simulink model "ASM_Traffic_new"  (R2024a)
settings: Solver=ode1  StartTime=SIM.tstart.v  StopTime=SIM.tend.v  FixedStep=SIM.StepSize.v  RelTol=1e-3
PostLoadFcn:
  | if any(exist('dsrtsu_mdlpostloadfcn', 'file') ~= 0), dsrtsu_mdlpostloadfcn('Execute', bdroot); end
  | try, asm_mdl_postloadfcn(bdroot, 'UpdateModel', 3600); catch, disp(lasterr); end,
InitFcn:
  | , if any(exist('rtifpga_mdlclblib', 'file') ~= 0), rtifpga_mdlclblib('Init', bdroot); end,
  | , if any(exist('dsmpb_private', 'file') ~= 0), dsmpb_private('dsmpb_mdlclblib', 'Init', bdroot); end,
undefined symbols (not defined in the file): _to_, a0b2, ASM_BrakeHydraulics_DemoSystems, ASM_VehicleDynamics_DemoSystems, b98103fe8ad365046cd0, BrakeCircuit, CPT, Crankshaft, DiscIntNeverNeededParam, dsmsi, FinalDriveAssembly, MDL, ModeSignals, Pos_BrakePedal_Maneuver, rad, RefSignals, s_to_rpm, SIM, SoftECU, Suspension, Tire, Transmission
libraries: ASM_Traffic_lib x135, simulink x100, ASM_Utils_lib x77, ASM_VehicleDynamics_lib x70, ASM_Environment_lib x22, dsmpblib x20, dsmsilib x15, MDLD_Utils_lib x10, ASM_BrakeHydraulics_lib x3
(part 17 of 63)

== system ASM_Traffic_new/AnimationInterface/ANIMATION_INTERFACE/Bounding_Boxes/BoundingBox_4 ==
  Index[] : Inport
  BoundigBoxes_Animation : Inport  Port=2
  Bus Selector : BusSelector  OutputSignals=Pos_x_CoorSysE[m],Pos_y_CoorSysE[m],Pos_z_CoorSysE[m],Angle_z_Objects_CoorSysE[deg],Angle_y_Objects_CoorSysE[deg],Angle_x_Objects_CoorSysE[deg],Length_Object[m],Width_Object[m],Height_Object[m]
  Mux : Mux  Inputs=3
  Mux1 : Mux  Inputs=3
  Mux2 : Mux  Inputs=3
  Selector{1..9} (9 alike) : Selector  IndexOptions=Index vector (port)  Indices=[1 3]  OutputSizes=1
  Pos_CoorSysE[m] : Outport  VectorParamsAs1DForOutWhenUnconnected=off
  Angle_CoorSysE[m] : Outport  Port=2  VectorParamsAs1DForOutWhenUnconnected=off
  Dimensions[m] : Outport  Port=3  VectorParamsAs1DForOutWhenUnconnected=off
  wires:
  Bus Selector/9 -> Selector9/1  "<Height_Object[m]>"
  Bus Selector/8 -> Selector8/1  "<Width_Object[m]>"
  Bus Selector/7 -> Selector6/1  "<Length_Object[m]>"
  Bus Selector/6 -> Selector7/1  "<Angle_x_Objects_CoorSysE[deg]>"
  Bus Selector/5 -> Selector5/1  "<Angle_y_Objects_CoorSysE[deg]>"
  Bus Selector/4 -> Selector4/1  "<Angle_z_Objects_CoorSysE[deg]>"
  Bus Selector/3 -> Selector3/1  "<Pos_z_CoorSysE[m]>"
  Bus Selector/2 -> Selector2/1  "<Pos_y_CoorSysE[m]>"
  Bus Selector/1 -> Selector1/1  "<Pos_x_CoorSysE[m]>"
  BoundigBoxes_Animation/1 -> Bus Selector/1
  Selector5/1 -> Mux1/2
  Mux1/1 -> Angle_CoorSysE[m]/1
  Mux/1 -> Pos_CoorSysE[m]/1
  Index[]/1 -> Selector3/2, Selector4/2, Selector9/2, Selector8/2, Selector6/2, Selector7/2, Selector5/2, Selector2/2, Selector1/2
  Selector1/1 -> Mux/1
  Selector2/1 -> Mux/2
  Selector3/1 -> Mux/3
  Selector7/1 -> Mux1/3
  Selector4/1 -> Mux1/1
  Selector6/1 -> Mux2/1
  Selector8/1 -> Mux2/2
  Selector9/1 -> Mux2/3
  Mux2/1 -> Dimensions[m]/1

== system ASM_Traffic_new/AnimationInterface/ANIMATION_INTERFACE/Bounding_Boxes/BoundingBox_5 ==
  Index[] : Inport
  BoundigBoxes_Animation : Inport  Port=2
  Bus Selector : BusSelector  OutputSignals=Pos_x_CoorSysE[m],Pos_y_CoorSysE[m],Pos_z_CoorSysE[m],Angle_z_Objects_CoorSysE[deg],Angle_y_Objects_CoorSysE[deg],Angle_x_Objects_CoorSysE[deg],Length_Object[m],Width_Object[m],Height_Object[m]
  Mux : Mux  Inputs=3
  Mux1 : Mux  Inputs=3
  Mux2 : Mux  Inputs=3
  Selector{1..9} (9 alike) : Selector  IndexOptions=Index vector (port)  Indices=[1 3]  OutputSizes=1
  Pos_CoorSysE[m] : Outport  VectorParamsAs1DForOutWhenUnconnected=off
  Angle_CoorSysE[m] : Outport  Port=2  VectorParamsAs1DForOutWhenUnconnected=off
  Dimensions[m] : Outport  Port=3  VectorParamsAs1DForOutWhenUnconnected=off
  wires:
  Mux2/1 -> Dimensions[m]/1
  Selector9/1 -> Mux2/3
  Selector8/1 -> Mux2/2
  Selector6/1 -> Mux2/1
  Selector4/1 -> Mux1/1
  Selector7/1 -> Mux1/3
  Selector3/1 -> Mux/3
  Selector2/1 -> Mux/2
  Selector1/1 -> Mux/1
  Index[]/1 -> Selector1/2, Selector2/2, Selector5/2, Selector7/2, Selector6/2, Selector8/2, Selector9/2, Selector4/2, Selector3/2
  Mux/1 -> Pos_CoorSysE[m]/1
  Mux1/1 -> Angle_CoorSysE[m]/1
  Selector5/1 -> Mux1/2
  BoundigBoxes_Animation/1 -> Bus Selector/1
  Bus Selector/1 -> Selector1/1  "<Pos_x_CoorSysE[m]>"
  Bus Selector/2 -> Selector2/1  "<Pos_y_CoorSysE[m]>"
  Bus Selector/3 -> Selector3/1  "<Pos_z_CoorSysE[m]>"
  Bus Selector/4 -> Selector4/1  "<Angle_z_Objects_CoorSysE[deg]>"
  Bus Selector/5 -> Selector5/1  "<Angle_y_Objects_CoorSysE[deg]>"
  Bus Selector/6 -> Selector7/1  "<Angle_x_Objects_CoorSysE[deg]>"
  Bus Selector/7 -> Selector6/1  "<Length_Object[m]>"
  Bus Selector/8 -> Selector8/1  "<Width_Object[m]>"
  Bus Selector/9 -> Selector9/1  "<Height_Object[m]>"

== system ASM_Traffic_new/AnimationInterface/ANIMATION_INTERFACE/Bounding_Boxes/BoundingBox_6 ==
  Index[] : Inport
  BoundigBoxes_Animation : Inport  Port=2
  Bus Selector : BusSelector  OutputSignals=Pos_x_CoorSysE[m],Pos_y_CoorSysE[m],Pos_z_CoorSysE[m],Angle_z_Objects_CoorSysE[deg],Angle_y_Objects_CoorSysE[deg],Angle_x_Objects_CoorSysE[deg],Length_Object[m],Width_Object[m],Height_Object[m]
  Mux : Mux  Inputs=3
  Mux1 : Mux  Inputs=3
  Mux2 : Mux  Inputs=3
  Selector{1..9} (9 alike) : Selector  IndexOptions=Index vector (port)  Indices=[1 3]  OutputSizes=1
  Pos_CoorSysE[m] : Outport  VectorParamsAs1DForOutWhenUnconnected=off
  Angle_CoorSysE[m] : Outport  Port=2  VectorParamsAs1DForOutWhenUnconnected=off
  Dimensions[m] : Outport  Port=3  VectorParamsAs1DForOutWhenUnconnected=off
  wires:
  Bus Selector/9 -> Selector9/1  "<Height_Object[m]>"
  Bus Selector/8 -> Selector8/1  "<Width_Object[m]>"
  Bus Selector/7 -> Selector6/1  "<Length_Object[m]>"
  Bus Selector/6 -> Selector7/1  "<Angle_x_Objects_CoorSysE[deg]>"
  Bus Selector/5 -> Selector5/1  "<Angle_y_Objects_CoorSysE[deg]>"
  Bus Selector/4 -> Selector4/1  "<Angle_z_Objects_CoorSysE[deg]>"
  Bus Selector/3 -> Selector3/1  "<Pos_z_CoorSysE[m]>"
  Bus Selector/2 -> Selector2/1  "<Pos_y_CoorSysE[m]>"
  Bus Selector/1 -> Selector1/1  "<Pos_x_CoorSysE[m]>"
  BoundigBoxes_Animation/1 -> Bus Selector/1
  Selector5/1 -> Mux1/2
  Mux1/1 -> Angle_CoorSysE[m]/1
  Mux/1 -> Pos_CoorSysE[m]/1
  Index[]/1 -> Selector3/2, Selector4/2, Selector9/2, Selector8/2, Selector6/2, Selector7/2, Selector5/2, Selector2/2, Selector1/2
  Selector1/1 -> Mux/1
  Selector2/1 -> Mux/2
  Selector3/1 -> Mux/3
  Selector7/1 -> Mux1/3
  Selector4/1 -> Mux1/1
  Selector6/1 -> Mux2/1
  Selector8/1 -> Mux2/2
  Selector9/1 -> Mux2/3
  Mux2/1 -> Dimensions[m]/1

== system ASM_Traffic_new/AnimationInterface/ANIMATION_INTERFACE/Bounding_Boxes/BoundingBox_7 ==
  Index[] : Inport
  BoundigBoxes_Animation : Inport  Port=2
  Bus Selector : BusSelector  OutputSignals=Pos_x_CoorSysE[m],Pos_y_CoorSysE[m],Pos_z_CoorSysE[m],Angle_z_Objects_CoorSysE[deg],Angle_y_Objects_CoorSysE[deg],Angle_x_Objects_CoorSysE[deg],Length_Object[m],Width_Object[m],Height_Object[m]
  Mux : Mux  Inputs=3
  Mux1 : Mux  Inputs=3
  Mux2 : Mux  Inputs=3
  Selector{1..9} (9 alike) : Selector  IndexOptions=Index vector (port)  Indices=[1 3]  OutputSizes=1
  Pos_CoorSysE[m] : Outport  VectorParamsAs1DForOutWhenUnconnected=off
  Angle_CoorSysE[m] : Outport  Port=2  VectorParamsAs1DForOutWhenUnconnected=off
  Dimensions[m] : Outport  Port=3  VectorParamsAs1DForOutWhenUnconnected=off
  wires:
  Bus Selector/9 -> Selector9/1  "<Height_Object[m]>"
  Bus Selector/8 -> Selector8/1  "<Width_Object[m]>"
  Bus Selector/7 -> Selector6/1  "<Length_Object[m]>"
  Bus Selector/6 -> Selector7/1  "<Angle_x_Objects_CoorSysE[deg]>"
  Bus Selector/5 -> Selector5/1  "<Angle_y_Objects_CoorSysE[deg]>"
  Bus Selector/4 -> Selector4/1  "<Angle_z_Objects_CoorSysE[deg]>"
  Bus Selector/3 -> Selector3/1  "<Pos_z_CoorSysE[m]>"
  Bus Selector/2 -> Selector2/1  "<Pos_y_CoorSysE[m]>"
  Bus Selector/1 -> Selector1/1  "<Pos_x_CoorSysE[m]>"
  BoundigBoxes_Animation/1 -> Bus Selector/1
  Selector5/1 -> Mux1/2
  Mux1/1 -> Angle_CoorSysE[m]/1
  Mux/1 -> Pos_CoorSysE[m]/1
  Index[]/1 -> Selector3/2, Selector4/2, Selector9/2, Selector8/2, Selector6/2, Selector7/2, Selector5/2, Selector2/2, Selector1/2
  Selector1/1 -> Mux/1
  Selector2/1 -> Mux/2
  Selector3/1 -> Mux/3
  Selector7/1 -> Mux1/3
  Selector4/1 -> Mux1/1
  Selector6/1 -> Mux2/1
  Selector8/1 -> Mux2/2
  Selector9/1 -> Mux2/3
  Mux2/1 -> Dimensions[m]/1

== system ASM_Traffic_new/AnimationInterface/ANIMATION_INTERFACE/Bounding_Boxes/BoundingBox_8 ==
  Index[] : Inport
  BoundigBoxes_Animation : Inport  Port=2
  Bus Selector : BusSelector  OutputSignals=Pos_x_CoorSysE[m],Pos_y_CoorSysE[m],Pos_z_CoorSysE[m],Angle_z_Objects_CoorSysE[deg],Angle_y_Objects_CoorSysE[deg],Angle_x_Objects_CoorSysE[deg],Length_Object[m],Width_Object[m],Height_Object[m]
  Mux : Mux  Inputs=3
  Mux1 : Mux  Inputs=3
  Mux2 : Mux  Inputs=3
  Selector{1..9} (9 alike) : Selector  IndexOptions=Index vector (port)  Indices=[1 3]  OutputSizes=1
  Pos_CoorSysE[m] : Outport  VectorParamsAs1DForOutWhenUnconnected=off
  Angle_CoorSysE[m] : Outport  Port=2  VectorParamsAs1DForOutWhenUnconnected=off
  Dimensions[m] : Outport  Port=3  VectorParamsAs1DForOutWhenUnconnected=off
  wires:
  Mux2/1 -> Dimensions[m]/1
  Selector9/1 -> Mux2/3
  Selector8/1 -> Mux2/2
  Selector6/1 -> Mux2/1
  Selector4/1 -> Mux1/1
  Selector7/1 -> Mux1/3
  Selector3/1 -> Mux/3
  Selector2/1 -> Mux/2
  Selector1/1 -> Mux/1
  Index[]/1 -> Selector1/2, Selector2/2, Selector5/2, Selector7/2, Selector6/2, Selector8/2, Selector9/2, Selector4/2, Selector3/2
  Mux/1 -> Pos_CoorSysE[m]/1
  Mux1/1 -> Angle_CoorSysE[m]/1
  Selector5/1 -> Mux1/2
  BoundigBoxes_Animation/1 -> Bus Selector/1
  Bus Selector/1 -> Selector1/1  "<Pos_x_CoorSysE[m]>"
  Bus Selector/2 -> Selector2/1  "<Pos_y_CoorSysE[m]>"
  Bus Selector/3 -> Selector3/1  "<Pos_z_CoorSysE[m]>"
  Bus Selector/4 -> Selector4/1  "<Angle_z_Objects_CoorSysE[deg]>"
  Bus Selector/5 -> Selector5/1  "<Angle_y_Objects_CoorSysE[deg]>"
  Bus Selector/6 -> Selector7/1  "<Angle_x_Objects_CoorSysE[deg]>"
  Bus Selector/7 -> Selector6/1  "<Length_Object[m]>"
  Bus Selector/8 -> Selector8/1  "<Width_Object[m]>"
  Bus Selector/9 -> Selector9/1  "<Height_Object[m]>"

== system ASM_Traffic_new/AnimationInterface/ANIMATION_INTERFACE/Bounding_Boxes/BoundingBox_9 ==
  Index[] : Inport
  BoundigBoxes_Animation : Inport  Port=2
  Bus Selector : BusSelector  OutputSignals=Pos_x_CoorSysE[m],Pos_y_CoorSysE[m],Pos_z_CoorSysE[m],Angle_z_Objects_CoorSysE[deg],Angle_y_Objects_CoorSysE[deg],Angle_x_Objects_CoorSysE[deg],Length_Object[m],Width_Object[m],Height_Object[m]
  Mux : Mux  Inputs=3
  Mux1 : Mux  Inputs=3
  Mux2 : Mux  Inputs=3
  Selector{1..9} (9 alike) : Selector  IndexOptions=Index vector (port)  Indices=[1 3]  OutputSizes=1
  Pos_CoorSysE[m] : Outport  VectorParamsAs1DForOutWhenUnconnected=off
  Angle_CoorSysE[m] : Outport  Port=2  VectorParamsAs1DForOutWhenUnconnected=off
  Dimensions[m] : Outport  Port=3  VectorParamsAs1DForOutWhenUnconnected=off
  wires:
  Mux2/1 -> Dimensions[m]/1
  Selector9/1 -> Mux2/3
  Selector8/1 -> Mux2/2
  Selector6/1 -> Mux2/1
  Selector4/1 -> Mux1/1
  Selector7/1 -> Mux1/3
  Selector3/1 -> Mux/3
  Selector2/1 -> Mux/2
  Selector1/1 -> Mux/1
  Index[]/1 -> Selector1/2, Selector2/2, Selector5/2, Selector7/2, Selector6/2, Selector8/2, Selector9/2, Selector4/2, Selector3/2
  Mux/1 -> Pos_CoorSysE[m]/1
  Mux1/1 -> Angle_CoorSysE[m]/1
  Selector5/1 -> Mux1/2
  BoundigBoxes_Animation/1 -> Bus Selector/1
  Bus Selector/1 -> Selector1/1  "<Pos_x_CoorSysE[m]>"
  Bus Selector/2 -> Selector2/1  "<Pos_y_CoorSysE[m]>"
  Bus Selector/3 -> Selector3/1  "<Pos_z_CoorSysE[m]>"
  Bus Selector/4 -> Selector4/1  "<Angle_z_Objects_CoorSysE[deg]>"
  Bus Selector/5 -> Selector5/1  "<Angle_y_Objects_CoorSysE[deg]>"
  Bus Selector/6 -> Selector7/1  "<Angle_x_Objects_CoorSysE[deg]>"
  Bus Selector/7 -> Selector6/1  "<Length_Object[m]>"
  Bus Selector/8 -> Selector8/1  "<Width_Object[m]>"
  Bus Selector/9 -> Selector9/1  "<Height_Object[m]>"

== system ASM_Traffic_new/AnimationInterface/ANIMATION_INTERFACE/Bounding_Boxes/EnableBoxVisualization ==
  Environment_Animation : Inport
  Bus Creator : BusCreator  Inputs=9
  Bus Selector : BusSelector  OutputSignals=Boundingbox_DetectedObjects.Pos_x_CoorSysE[m],Boundingbox_DetectedObjects.Pos_y_CoorSysE[m],Boundingbox_DetectedObjects.Pos_z_CoorSysE[m],Boundingbox_DetectedObjects.Angle_x_Objects_CoorSysE[deg],Boundingbox_DetectedObjects.Angle_y_Objects_CoorSysE[deg],Boundingbox_DetectedObjects.Angle_z_Objects_CoorSysE[deg],Boundingbox_DetectedObjects.Length_Object[m],Boundingbox_DetectedObjects.Width_Object[m],Boundingbox_DetectedObjects.Height_Object[m]
  Constant : Constant  Value=zeros(1,10)
  Enable_BoxVisualization[0|1] : Constant  Value=[1 1 1 1 1 1 1 1 1 1]
  Move_Unused_Bounding_Boxes : MATLAB Function  TreatAsAtomicUnit=on
  Multiport Switch : MultiPortSwitch  DataPortOrder=Zero-based contiguous  Inputs=2  zeroidx=on  SaturateOnIntegerOverflow=off  InputSameDT=off
  Multiport Switch1 : MultiPortSwitch  DataPortOrder=Zero-based contiguous  Inputs=2  zeroidx=on  SaturateOnIntegerOverflow=off  InputSameDT=off
  Multiport Switch2 : MultiPortSwitch  DataPortOrder=Zero-based contiguous  Inputs=2  zeroidx=on  SaturateOnIntegerOverflow=off  InputSameDT=off
  BoundigBoxes_Animation : Outport  VectorParamsAs1DForOutWhenUnconnected=off
  wires:
  Bus Selector/9 -> Move_Unused_Bounding_Boxes/9(height_in)  "<Height_Object[m]>"
  Bus Selector/8 -> Move_Unused_Bounding_Boxes/8(width_in)  "<Width_Object[m]>"
  Bus Selector/7 -> Move_Unused_Bounding_Boxes/7(length_in)  "<Length_Object[m]>"
  Move_Unused_Bounding_Boxes/9(height_out) -> Bus Creator/9  "Height_Object[m]"
  Move_Unused_Bounding_Boxes/8(width_out) -> Bus Creator/8  "Width_Object[m]"
  Move_Unused_Bounding_Boxes/7(length_out) -> Bus Creator/7  "Length_Object[m]"
  Move_Unused_Bounding_Boxes/6(angle_z_out) -> Bus Creator/6  "Angle_z_Objects_CoorSysE[deg]"
  Move_Unused_Bounding_Boxes/5(angle_y_out) -> Bus Creator/5  "Angle_y_Objects_CoorSysE[deg]"
  Move_Unused_Bounding_Boxes/4(angle_x_out) -> Bus Creator/4  "Angle_x_Objects_CoorSysE[deg]"
  Move_Unused_Bounding_Boxes/3(pos_z_out) -> Bus Creator/3  "Pos_z_CoorSysE[m]"
  Move_Unused_Bounding_Boxes/2(pos_y_out) -> Bus Creator/2  "Pos_y_CoorSysE[m]"
  Move_Unused_Bounding_Boxes/1(pos_x_out) -> Bus Creator/1  "Pos_x_CoorSysE[m]"
  Bus Creator/1 -> BoundigBoxes_Animation/1
  Bus Selector/6 -> Move_Unused_Bounding_Boxes/6(angle_z_in)  "<Angle_z_Objects_CoorSysE[deg]>"
  Bus Selector/5 -> Move_Unused_Bounding_Boxes/5(angle_y_in)  "<Angle_y_Objects_CoorSysE[deg]>"
  Bus Selector/4 -> Move_Unused_Bounding_Boxes/4(angle_x_in)  "<Angle_x_Objects_CoorSysE[deg]>"
  Bus Selector/3 -> Multiport Switch2/3  "<Pos_z_CoorSysE[m]>"
  Bus Selector/2 -> Multiport Switch1/3  "<Pos_y_CoorSysE[m]>"
  Bus Selector/1 -> Multiport Switch/3  "<Pos_x_CoorSysE[m]>"
  Environment_Animation/1 -> Bus Selector/1
  Constant/1 -> Multiport Switch/2, Multiport Switch1/2, Multiport Switch2/2
  Enable_BoxVisualization[0|1]/1 -> Multiport Switch/1, Multiport Switch1/1, Multiport Switch2/1
  Multiport Switch2/1 -> Move_Unused_Bounding_Boxes/3(pos_z_in)  "Pos_z_CoorSysE[m]"
  Multiport Switch1/1 -> Move_Unused_Bounding_Boxes/2(pos_y_in)  "Pos_y_CoorSysE[m]"
  Multiport Switch/1 -> Move_Unused_Bounding_Boxes/1(pos_x_in)  "Pos_x_CoorSysE[m]"

== system ASM_Traffic_new/AnimationInterface/ANIMATION_INTERFACE/Connection_Settings/Communication_Service ==
  Tx_Length : Inport
  Tx_Data : Inport  Port=2
  ReferenceTime[s] : Inport  Port=3
  Reset[0|1] : Inport  Port=4
  Connected_ : Constant  OutDataTypeStr=Inherit: Inherit via back propagation
  Display : Display
      settings: Format=decimal (Stored Integer)
  Rx_Data_ : Constant  Value=zeros(65507,1)  OutDataTypeStr=Inherit: Inherit via back propagation
  Rx_Length_ : Constant  Value=0  OutDataTypeStr=Inherit: Inherit via back propagation
  dsmsi_communication_service_BL1 : dsmsilib/dsmsi_communication_service_BL1  TypeOfData=Animation (Topic ID 1004)  ModelStepSize=ModelStepSize  NumSamples=NumSamples  MaxMessageSize=MaxMessageSize  blockVersion=60
      settings: SourceProductName=dSPACE MSI Blockset
  Connected : Outport
  Tx_Sent_bytes : Outport  Port=2
  Rx_Length : Outport  Port=3
  Rx_Data : Outport  Port=4
  wires:
  ReferenceTime[s]/1 -> dsmsi_communication_service_BL1/3
  Reset[0|1]/1 -> dsmsi_communication_service_BL1/4
  Rx_Data_/1 -> Rx_Data/1
  Rx_Length_/1 -> Rx_Length/1
  Connected_/1 -> Connected/1
  dsmsi_communication_service_BL1/2 -> Tx_Sent_bytes/1
  dsmsi_communication_service_BL1/1 -> Display/1
  Tx_Length/1 -> dsmsi_communication_service_BL1/1
  Tx_Data/1 -> dsmsi_communication_service_BL1/2

== system ASM_Traffic_new/AnimationInterface/ANIMATION_INTERFACE/Connection_Settings/Communication_Service_Common_Signals ==
  Environment_Animation : Inport
  Bus Selector : BusSelector  OutputSignals=ManeuverTime[s],ManeuverState[]
  Data Type Conversion : DataTypeConversion  OutDataTypeStr=uint8  SaturateOnIntegerOverflow=off  RndMeth=Floor
  Init : simulink/Logic and Bit Operations/Compare To Constant  relop===  const=2  OutDataTypeStr=boolean
  ReferenceTime[s] : Outport
  Reset[0|1] : Outport  Port=2
  wires:
  Bus Selector/2 -> Init/1  "<ManeuverState[]>"
  Data Type Conversion/1 -> Reset[0|1]/1
  Init/1 -> Data Type Conversion/1
  Environment_Animation/1 -> Bus Selector/1
  Bus Selector/1 -> ReferenceTime[s]/1  "<ManeuverTime[s]>"

== system ASM_Traffic_new/AnimationInterface/ANIMATION_INTERFACE/Connection_Settings/Ethernet_TCP ==
  Tx_Length : Inport
  Tx_Data : Inport  Port=2
  HIL : Subsystem  Commented=on
  MultiportSwitch{,1..3} (4 alike) : MultiPortSwitch  DataPortOrder=Zero-based contiguous  Inputs=2  zeroidx=on  SaturateOnIntegerOverflow=off  InputSameDT=off
  SIL : Subsystem  Tag=AnimationInterface_SIL
  Sw_Mode[0SIL|1HIL] : Constant  Value=Sw_Mode
  Connected : Outport
  Tx_Sent_bytes : Outport  Port=2
  Rx_Length : Outport  Port=3
  Rx_Data : Outport  Port=4
  wires:
  MultiportSwitch1/1 -> Tx_Sent_bytes/1
  MultiportSwitch2/1 -> Rx_Length/1
  MultiportSwitch3/1 -> Rx_Data/1
  MultiportSwitch/1 -> Connected/1
  Sw_Mode[0SIL|1HIL]/1 -> MultiportSwitch/1, MultiportSwitch1/1, MultiportSwitch2/1, MultiportSwitch3/1
  HIL/4(Rx_Data) -> MultiportSwitch3/3
  SIL/4(Rx_Data) -> MultiportSwitch3/2
  HIL/3(Rx_Length) -> MultiportSwitch2/3
  SIL/3(Rx_Length) -> MultiportSwitch2/2
  HIL/2(Tx_Sent_bytes) -> MultiportSwitch1/3
  SIL/2(Tx_Sent_bytes) -> MultiportSwitch1/2
  HIL/1(Connected) -> MultiportSwitch/3
  SIL/1(Connected) -> MultiportSwitch/2
  Tx_Length/1 -> SIL/1(Tx_Length), HIL/1(Tx_Length)
  Tx_Data/1 -> SIL/2(Tx_Data), HIL/2(Tx_Data)

== system ASM_Traffic_new/AnimationInterface/ANIMATION_INTERFACE/Fellows/Fellow_Rotation ==
  In : Inport
  Bus Selector : BusSelector  OutputSignals=Angle_Yaw_Fellows[deg],Angle_Pitch_Fellows[deg],Angle_Roll_Fellows[deg]
  Reshape3 : Reshape
  Transpose2 : Math  Operator=transpose
  Vector Concatenate1 : Concatenate  NumInputs=3  Mode=Multidimensional array  ConcatenateDimension=2
  Out : Outport
  wires:
  Transpose2/1 -> Reshape3/1
  Bus Selector/2 -> Vector Concatenate1/2  "<Angle_Pitch_Fellows[deg]>"
  Bus Selector/3 -> Vector Concatenate1/3  "<Angle_Roll_Fellows[deg]>"
  Vector Concatenate1/1 -> Transpose2/1
  Bus Selector/1 -> Vector Concatenate1/1  "<Angle_Yaw_Fellows[deg]>"
  Reshape3/1 -> Out/1
  In/1 -> Bus Selector/1

== system ASM_Traffic_new/AnimationInterface/ANIMATION_INTERFACE/Fellows/Fellow_Scaling ==
  In : Inport
  Reshape4 : Reshape
  Transpose3 : Math  Operator=transpose
  Vector Concatenate2 : Concatenate  NumInputs=3  Mode=Multidimensional array  ConcatenateDimension=2
  Out : Outport
  wires:
  Reshape4/1 -> Out/1
  Vector Concatenate2/1 -> Transpose3/1
  Transpose3/1 -> Reshape4/1
  In/1 -> Vector Concatenate2/1, Vector Concatenate2/2, Vector Concatenate2/3

== system ASM_Traffic_new/AnimationInterface/ANIMATION_INTERFACE/Fellows/Fellow_Translation ==
  In : Inport
  Bus Selector1 : BusSelector  OutputSignals=Pos_x_Fellows[m],Pos_y_Fellows[m],Pos_z_Fellows[m]
  Reshape2 : Reshape
  Transpose1 : Math  Operator=transpose
  Vector Concatenate : Concatenate  NumInputs=3  Mode=Multidimensional array  ConcatenateDimension=2
  Out : Outport
  wires:
  In/1 -> Bus Selector1/1
  Reshape2/1 -> Out/1
  Bus Selector1/3 -> Vector Concatenate/3  "<Pos_z_Fellows[m]>"
  Bus Selector1/2 -> Vector Concatenate/2  "<Pos_y_Fellows[m]>"
  Bus Selector1/1 -> Vector Concatenate/1  "<Pos_x_Fellows[m]>"
  Transpose1/1 -> Reshape2/1
  Vector Concatenate/1 -> Transpose1/1

== system ASM_Traffic_new/AnimationInterface/ANIMATION_INTERFACE/Lane_Sensor/Sensor_L_Rotation ==
  Sw_Pitch_Angle_Offset : Inport
  In : Inport  Port=2
  Constant1 : Constant  Value=90
  Constant2 : Constant  Value=0
  Constant3 : Constant  Value=0
  Multiport Switch : MultiPortSwitch  DataPortOrder=Zero-based contiguous  Inputs=2  zeroidx=on  SaturateOnIntegerOverflow=off  InputSameDT=off
  Mux3 : Mux  Inputs=3
  Selector : Selector  IndexOptions=Index vector (dialog)  Indices=[1]  OutputSizes=1
  Out : Outport
  wires:
  Constant3/1 -> Mux3/3
  Multiport Switch/1 -> Mux3/2
  Constant1/1 -> Multiport Switch/3
  Constant2/1 -> Multiport Switch/2
  Sw_Pitch_Angle_Offset/1 -> Multiport Switch/1
  In/1 -> Selector/1
  Selector/1 -> Mux3/1
  Mux3/1 -> Out/1

== system ASM_Traffic_new/AnimationInterface/ANIMATION_INTERFACE/Lane_Sensor/Sensor_L_Scaling ==
  In : Inport
  CastToDouble : DataTypeConversion  OutDataTypeStr=double  SaturateOnIntegerOverflow=off  RndMeth=Floor
  Compare To Zero : simulink/Logic and Bit Operations/Compare To Zero  relop=~=  OutDataTypeStr=uint8
  Mux : Mux  Inputs=3
  Selector : Selector  IndexOptions=Index vector (dialog)  Indices=[1]  OutputSizes=1
  Out : Outport
  wires:
  In/1 -> Selector/1
  Mux/1 -> Out/1
  CastToDouble/1 -> Mux/1, Mux/2, Mux/3
  Selector/1 -> Compare To Zero/1
  Compare To Zero/1 -> CastToDouble/1

== system ASM_Traffic_new/AnimationInterface/ANIMATION_INTERFACE/Lane_Sensor/Sensor_L_Translation ==
  In : Inport
  Bus to Vector : BusToVector
  Demux : Demux  Outputs=3
  Mux2 : Mux  Inputs=3
  Selector1 : Selector  IndexOptions=Index vector (dialog)  Indices=[1]  OutputSizes=1
  Selector2 : Selector  IndexOptions=Index vector (dialog)  Indices=[1]  OutputSizes=1
  Selector3 : Selector  IndexOptions=Index vector (dialog)  Indices=[1]  OutputSizes=1
  Out : Outport
  wires:
  In/1 -> Bus to Vector/1
  Demux/2 -> Selector2/1
  Selector1/1 -> Mux2/1
  Demux/1 -> Selector1/1
  Demux/3 -> Selector3/1
  Bus to Vector/1 -> Demux/1
  Selector2/1 -> Mux2/2
  Selector3/1 -> Mux2/3
  Mux2/1 -> Out/1

== system ASM_Traffic_new/AnimationInterface/ANIMATION_INTERFACE/Lane_Sensor/Sensor_R_Rotation ==
  Sw_Pitch_Angle_Offset : Inport
  In : Inport  Port=2
  Constant1 : Constant  Value=90
  Constant2 : Constant  Value=0
  Constant3 : Constant  Value=0
  Multiport Switch : MultiPortSwitch  DataPortOrder=Zero-based contiguous  Inputs=2  zeroidx=on  SaturateOnIntegerOverflow=off  InputSameDT=off
  Mux3 : Mux  Inputs=3
  Selector : Selector  IndexOptions=Index vector (dialog)  Indices=[1]  OutputSizes=1
  Out : Outport
  wires:
  Mux3/1 -> Out/1
  Multiport Switch/1 -> Mux3/2
  Constant2/1 -> Multiport Switch/2
  Selector/1 -> Mux3/1
  In/1 -> Selector/1
  Constant3/1 -> Mux3/3
  Constant1/1 -> Multiport Switch/3
  Sw_Pitch_Angle_Offset/1 -> Multiport Switch/1

== system ASM_Traffic_new/AnimationInterface/ANIMATION_INTERFACE/Lane_Sensor/Sensor_R_Scaling ==
  In : Inport
  CastToDouble : DataTypeConversion  OutDataTypeStr=double  SaturateOnIntegerOverflow=off  RndMeth=Floor
  Compare To Zero : simulink/Logic and Bit Operations/Compare To Zero  relop=~=  OutDataTypeStr=uint8
  Mux : Mux  Inputs=3
  Selector : Selector  IndexOptions=Index vector (dialog)  Indices=[1]  OutputSizes=1
  Out : Outport
  wires:
  Compare To Zero/1 -> CastToDouble/1
  Selector/1 -> Compare To Zero/1
  CastToDouble/1 -> Mux/3, Mux/2, Mux/1
  Mux/1 -> Out/1
  In/1 -> Selector/1

== system ASM_Traffic_new/AnimationInterface/ANIMATION_INTERFACE/Lane_Sensor/Sensor_R_Translation ==
  In : Inport
  Bus to Vector : BusToVector
  Demux : Demux  Outputs=3
  Mux2 : Mux  Inputs=3
  Selector1 : Selector  IndexOptions=Index vector (dialog)  Indices=[1]  OutputSizes=1
  Selector2 : Selector  IndexOptions=Index vector (dialog)  Indices=[1]  OutputSizes=1
  Selector3 : Selector  IndexOptions=Index vector (dialog)  Indices=[1]  OutputSizes=1
  Out : Outport
  wires:
  Mux2/1 -> Out/1
  Selector3/1 -> Mux2/3
  Selector2/1 -> Mux2/2
  Bus to Vector/1 -> Demux/1
  Demux/3 -> Selector3/1
  Demux/1 -> Selector1/1
  Selector1/1 -> Mux2/1
  Demux/2 -> Selector2/1
  In/1 -> Bus to Vector/1

== system ASM_Traffic_new/AnimationInterface/ANIMATION_INTERFACE/Lane_Sensor_Dynamic_Instruments/CalcLDWState ==
  NetworkItemType[] : Inport
  Dist_L[m] : Inport  Port=2
  Dist_R[m] : Inport  Port=3
  AND : Logic  IconShape=distinctive  AllPortsSameDT=off  OutDataTypeStr=boolean
  Compare To Constant1 : simulink/Logic and Bit Operations/Compare To Constant  relop=<=  const=0.01  OutDataTypeStr=boolean
  Compare To Constant2 : simulink/Logic and Bit Operations/Compare To Constant  relop=<=  const=0.2  OutDataTypeStr=boolean
  Compare To Constant3 : simulink/Logic and Bit Operations/Compare To Constant  relop=>  const=0.01  OutDataTypeStr=boolean
  Demux : Demux  Outputs=2
  Junction : Constant  Value=0  OutDataTypeStr=Inherit: Inherit via back propagation
  JunctionType : simulink/Logic and Bit Operations/Compare To Constant  relop===  const=3  OutDataTypeStr=boolean
  Mux : Mux  Inputs=2
  One : Constant  OutDataTypeStr=Inherit: Inherit via back propagation
  Switch : Switch  Criteria=u2 ~= 0  SaturateOnIntegerOverflow=off  InputSameDT=off
  Switch1 : Switch  Criteria=u2 ~= 0  SaturateOnIntegerOverflow=off  InputSameDT=off
  Switch2 : Switch  Criteria=u2 ~= 0  SaturateOnIntegerOverflow=off  InputSameDT=off
  Three : Constant  Value=3  OutDataTypeStr=Inherit: Inherit via back propagation
  Two : Constant  Value=2  OutDataTypeStr=Inherit: Inherit via back propagation
  LDWState_L[] : Outport  VectorParamsAs1DForOutWhenUnconnected=off
  LDWState_R[] : Outport  Port=2  VectorParamsAs1DForOutWhenUnconnected=off
  wires:
  Switch2/1 -> Demux/1
  Junction/1 -> Switch2/1
  JunctionType/1 -> Switch2/2
  Dist_R[m]/1 -> Mux/2
  Dist_L[m]/1 -> Mux/1
  Mux/1 -> Compare To Constant1/1, Compare To Constant2/1, Compare To Constant3/1
  Switch/1 -> Switch2/3
  Two/1 -> Switch1/1
  Switch1/1 -> Switch/3
  Three/1 -> Switch1/3
  AND/1 -> Switch1/2
  One/1 -> Switch/1
  Compare To Constant1/1 -> Switch/2
  Compare To Constant2/1 -> AND/2
  Compare To Constant3/1 -> AND/1
  NetworkItemType[]/1 -> JunctionType/1
  Demux/1 -> LDWState_L[]/1
  Demux/2 -> LDWState_R[]/1

== system ASM_Traffic_new/AnimationInterface/ANIMATION_INTERFACE/Sensors/Line_Sensor_Junction_Border_Points ==
  ModelSignals : Inport
  Bus Selector : BusSelector  OutputSignals=Pos_x_Junction_Border_Animation_CoorSys_E,Pos_y_Junction_Border_Animation_CoorSys_E,Pos_z_Junction_Border_Animation_CoorSys_E
  CC : Concatenate  NumInputs=3  Mode=Multidimensional array
  Reshape1 : Reshape  OutputDimensionality=Row vector (2-D)
  Reshape2 : Reshape  OutputDimensionality=Row vector (2-D)
  Reshape3 : Reshape  OutputDimensionality=Row vector (2-D)
  AnimationSignals : Outport  VectorParamsAs1DForOutWhenUnconnected=off
  wires:
  Reshape3/1 -> CC/3
  Reshape2/1 -> CC/2
  Reshape1/1 -> CC/1
  Bus Selector/3 -> Reshape3/1  "<Pos_z_Junction_Border_Animation_CoorSys_E>"
  Bus Selector/2 -> Reshape2/1  "<Pos_y_Junction_Border_Animation_CoorSys_E>"
  Bus Selector/1 -> Reshape1/1  "<Pos_x_Junction_Border_Animation_CoorSys_E>"
  CC/1 -> AnimationSignals/1
  ModelSignals/1 -> Bus Selector/1

== system ASM_Traffic_new/AnimationInterface/ANIMATION_INTERFACE/Sensors/Line_Sensor_Junction_Shape_ContObj_Points ==
  ModelSignals : Inport
  Bus Selector : BusSelector  OutputSignals=Pos_x_Junction_Shape_ContObj_Animation_CoorSys_E,Pos_y_Junction_Shape_ContObj_Animation_CoorSys_E,Pos_z_Junction_Shape_ContObj_Animation_CoorSys_E
  CC : Concatenate  NumInputs=3  Mode=Multidimensional array
  Reshape1 : Reshape  OutputDimensionality=Row vector (2-D)
  Reshape2 : Reshape  OutputDimensionality=Row vector (2-D)
  Reshape3 : Reshape  OutputDimensionality=Row vector (2-D)
  AnimationSignals : Outport  VectorParamsAs1DForOutWhenUnconnected=off
  wires:
  Reshape3/1 -> CC/3
  Reshape2/1 -> CC/2
  Reshape1/1 -> CC/1
  Bus Selector/3 -> Reshape3/1  "<Pos_z_Junction_Shape_ContObj_Animation_CoorSys_E>"
  Bus Selector/2 -> Reshape2/1  "<Pos_y_Junction_Shape_ContObj_Animation_CoorSys_E>"
  Bus Selector/1 -> Reshape1/1  "<Pos_x_Junction_Shape_ContObj_Animation_CoorSys_E>"
  CC/1 -> AnimationSignals/1
  ModelSignals/1 -> Bus Selector/1

== system ASM_Traffic_new/AnimationInterface/ANIMATION_INTERFACE/Sensors/Line_Sensor_Junction_Shape_Line_Points ==
  ModelSignals : Inport
  Bus Selector : BusSelector  OutputSignals=Pos_x_Junction_Shape_Line_Animation_CoorSys_E,Pos_y_Junction_Shape_Line_Animation_CoorSys_E,Pos_z_Junction_Shape_Line_Animation_CoorSys_E
  CC : Concatenate  NumInputs=3  Mode=Multidimensional array
  Reshape1 : Reshape  OutputDimensionality=Row vector (2-D)
  Reshape2 : Reshape  OutputDimensionality=Row vector (2-D)
  Reshape3 : Reshape  OutputDimensionality=Row vector (2-D)
  AnimationSignals : Outport  VectorParamsAs1DForOutWhenUnconnected=off
  wires:
  ModelSignals/1 -> Bus Selector/1
  CC/1 -> AnimationSignals/1
  Bus Selector/1 -> Reshape1/1  "<Pos_x_Junction_Shape_Line_Animation_CoorSys_E>"
  Bus Selector/2 -> Reshape2/1  "<Pos_y_Junction_Shape_Line_Animation_CoorSys_E>"
  Bus Selector/3 -> Reshape3/1  "<Pos_z_Junction_Shape_Line_Animation_CoorSys_E>"
  Reshape1/1 -> CC/1
  Reshape2/1 -> CC/2
  Reshape3/1 -> CC/3

== system ASM_Traffic_new/AnimationInterface/ANIMATION_INTERFACE/Sensors/Line_Sensor_Road_Lane_Points ==
  ModelSignals : Inport
  Bus Selector : BusSelector  OutputSignals=Pos_x_Road_Lane_Animation_CoorSys_E,Pos_y_Road_Lane_Animation_CoorSys_E,Pos_z_Road_Lane_Animation_CoorSys_E
  CC : Concatenate  NumInputs=3  Mode=Multidimensional array
  Reshape1 : Reshape  OutputDimensionality=Row vector (2-D)
  Reshape2 : Reshape  OutputDimensionality=Row vector (2-D)
  Reshape3 : Reshape  OutputDimensionality=Row vector (2-D)
  AnimationSignals : Outport  VectorParamsAs1DForOutWhenUnconnected=off
  wires:
  Reshape3/1 -> CC/3
  Reshape2/1 -> CC/2
  Reshape1/1 -> CC/1
  ModelSignals/1 -> Bus Selector/1
  CC/1 -> AnimationSignals/1
  Bus Selector/1 -> Reshape1/1  "<Pos_x_Road_Lane_Animation_CoorSys_E>"
  Bus Selector/2 -> Reshape2/1  "<Pos_y_Road_Lane_Animation_CoorSys_E>"
  Bus Selector/3 -> Reshape3/1  "<Pos_z_Road_Lane_Animation_CoorSys_E>"

== system ASM_Traffic_new/AnimationInterface/ANIMATION_INTERFACE/Sensors/Line_Sensor_Road_Shape_ContObj_Points ==
  ModelSignals : Inport
  Bus Selector : BusSelector  OutputSignals=Pos_x_Road_Shape_ContObj_Animation_CoorSys_E,Pos_y_Road_Shape_ContObj_Animation_CoorSys_E,Pos_z_Road_Shape_ContObj_Animation_CoorSys_E
  CC : Concatenate  NumInputs=3  Mode=Multidimensional array
  Reshape1 : Reshape  OutputDimensionality=Row vector (2-D)
  Reshape2 : Reshape  OutputDimensionality=Row vector (2-D)
  Reshape3 : Reshape  OutputDimensionality=Row vector (2-D)
  AnimationSignals : Outport  VectorParamsAs1DForOutWhenUnconnected=off
  wires:
  Reshape3/1 -> CC/3
  Reshape2/1 -> CC/2
  Reshape1/1 -> CC/1
  Bus Selector/3 -> Reshape3/1  "<Pos_z_Road_Shape_ContObj_Animation_CoorSys_E>"
  Bus Selector/2 -> Reshape2/1  "<Pos_y_Road_Shape_ContObj_Animation_CoorSys_E>"
  Bus Selector/1 -> Reshape1/1  "<Pos_x_Road_Shape_ContObj_Animation_CoorSys_E>"
  CC/1 -> AnimationSignals/1
  ModelSignals/1 -> Bus Selector/1

== system ASM_Traffic_new/AnimationInterface/ANIMATION_INTERFACE/Sensors/Line_Sensor_Road_Shape_Line_Points ==
  ModelSignals : Inport
  Bus Selector : BusSelector  OutputSignals=Pos_x_Road_Shape_Line_Animation_CoorSys_E,Pos_y_Road_Shape_Line_Animation_CoorSys_E,Pos_z_Road_Shape_Line_Animation_CoorSys_E
  CC : Concatenate  NumInputs=3  Mode=Multidimensional array
  Reshape1 : Reshape  OutputDimensionality=Row vector (2-D)
  Reshape2 : Reshape  OutputDimensionality=Row vector (2-D)
  Reshape3 : Reshape  OutputDimensionality=Row vector (2-D)
  AnimationSignals : Outport  VectorParamsAs1DForOutWhenUnconnected=off
  wires:
  Reshape3/1 -> CC/3
  Reshape2/1 -> CC/2
  Reshape1/1 -> CC/1
  ModelSignals/1 -> Bus Selector/1
  CC/1 -> AnimationSignals/1
  Bus Selector/1 -> Reshape1/1  "<Pos_x_Road_Shape_Line_Animation_CoorSys_E>"
  Bus Selector/2 -> Reshape2/1  "<Pos_y_Road_Shape_Line_Animation_CoorSys_E>"
  Bus Selector/3 -> Reshape3/1  "<Pos_z_Road_Shape_Line_Animation_CoorSys_E>"

== system ASM_Traffic_new/AnimationInterface/ANIMATION_INTERFACE/Sensors/Object_Sensor_2D_Points ==
  Transform_In : Inport
  Sw_Sensor_Selector[] : Inport  Port=2
  ObjectSensor2D_1_Animation : Inport  Port=3
  ObjectSensor2D_2_Animation : Inport  Port=4
  ObjectSensor2D_3_Animation : Inport  Port=5
  ObjectSensor2D_4_Animation : Inport  Port=6
  ObjectSensor2D_5_Animation : Inport  Port=7
  ObjectSensor2D_6_Animation : Inport  Port=8
  ObjectSensor2D_7_Animation : Inport  Port=9
  Calc_Object_Sensor_2D_Points : Subsystem
  Multiport Switch : MultiPortSwitch  Inputs=7  SaturateOnIntegerOverflow=off  InputSameDT=off
  Object_Sensor_2D_Transformation1 : Subsystem
  Saturation : Saturate  UpperLimit=7  LowerLimit=1
  AnimationSignals : Outport  VectorParamsAs1DForOutWhenUnconnected=off
  wires:
  Multiport Switch/1 -> Calc_Object_Sensor_2D_Points/2(ModelSignals), Object_Sensor_2D_Transformation1/2(ModelSignals)
  Sw_Sensor_Selector[]/1 -> Saturation/1
  ObjectSensor2D_1_Animation/1 -> Multiport Switch/2
  ObjectSensor2D_2_Animation/1 -> Multiport Switch/3
  ObjectSensor2D_3_Animation/1 -> Multiport Switch/4
  Calc_Object_Sensor_2D_Points/1(AnimationSignals) -> AnimationSignals/1
  Object_Sensor_2D_Transformation1/1(Transform_Out) -> Calc_Object_Sensor_2D_Points/1(Transform_In)
  Transform_In/1 -> Object_Sensor_2D_Transformation1/1(Transform_In1)
  ObjectSensor2D_4_Animation/1 -> Multiport Switch/5
  ObjectSensor2D_5_Animation/1 -> Multiport Switch/6
  ObjectSensor2D_6_Animation/1 -> Multiport Switch/7
  ObjectSensor2D_7_Animation/1 -> Multiport Switch/8
  Saturation/1 -> Multiport Switch/1

== system ASM_Traffic_new/AnimationInterface/ANIMATION_INTERFACE/Sensors/Object_Sensor_3D_CustomPoints ==
  Sw_Sensor_Selector[] : Inport
  ObjectSensor3D_1_CustomPoints_Animation : Inport  Port=2
  ObjectSensor3D_2_CustomPoints_Animation : Inport  Port=3
  ObjectSensor3D_3_CustomPoints_Animation : Inport  Port=4
  AdaptPointSensor1_To_Dim_60 : Subsystem
  AdaptPointSensor2_To_Dim_60 : Subsystem
  AdaptPointSensor3_To_Dim_60 : Subsystem
  Bus Selector3 : BusSelector  OutputSignals=ID[],Pos_CoorSys_E[x;y;z][m]
  Bus Selector5 : BusSelector  OutputSignals=ID[],Pos_CoorSys_E[x;y;z][m]
  Bus Selector8 : BusSelector  OutputSignals=ID[],Pos_CoorSys_E[x;y;z][m]
  Compare To Constant3 : simulink/Logic and Bit Operations/Compare To Constant  relop=>  const=-1  OutDataTypeStr=boolean
  DownAway_Dim_3_60 : Constant  Value=[zeros(60*2,1); zeros(60,1)-999999]
  Multiport Switch1 : MultiPortSwitch  SaturateOnIntegerOverflow=off  InputSameDT=off
  Multiport Switch2 : MultiPortSwitch  SaturateOnIntegerOverflow=off  InputSameDT=off
  Mux : Mux  Inputs=3
  Reshape_60_3 : Reshape  OutputDimensionality=Customize  OutputDimensions=[60,3]
  Saturation1 : Saturate  UpperLimit=3  LowerLimit=1
  Sw : MultiPortSwitch  DataPortOrder=Zero-based contiguous  Inputs=2  zeroidx=on  SaturateOnIntegerOverflow=off  InputSameDT=off
  Transpose : Math  Operator=transpose  SignedPower=on
  AnimationSignals : Outport  VectorParamsAs1DForOutWhenUnconnected=off
  wires:
  AdaptPointSensor2_To_Dim_60/1(ID_Adatpted[]) -> Multiport Switch2/3
  AdaptPointSensor2_To_Dim_60/2(Pos_ObjectPoint_CoorSys_E_Adapted[x;y;z][m]) -> Multiport Switch1/3
  Sw/1 -> Reshape_60_3/1
  Saturation1/1 -> Multiport Switch2/1, Multiport Switch1/1
  DownAway_Dim_3_60/1 -> Sw/2
  Sw_Sensor_Selector[]/1 -> Saturation1/1
  Compare To Constant3/1 -> Mux/1, Mux/2, Mux/3
  Mux/1 -> Sw/1
  Bus Selector8/1 -> AdaptPointSensor3_To_Dim_60/1(ID[])  "<ID[]>"
  AdaptPointSensor1_To_Dim_60/2(Pos_ObjectPoint_CoorSys_E_Adapted[x;y;z][m]) -> Multiport Switch1/2
  AdaptPointSensor1_To_Dim_60/1(ID_Adatpted[]) -> Multiport Switch2/2
  ObjectSensor3D_1_CustomPoints_Animation/1 -> Bus Selector3/1
  Bus Selector3/2 -> AdaptPointSensor1_To_Dim_60/2(Pos_ObjectPoint_CoorSys_E[x;y;z][m])  "<Pos_CoorSys_E[x;y;z][m]>"
  Bus Selector3/1 -> AdaptPointSensor1_To_Dim_60/1(ID[])  "<ID[]>"
  ObjectSensor3D_3_CustomPoints_Animation/1 -> Bus Selector8/1
  ObjectSensor3D_2_CustomPoints_Animation/1 -> Bus Selector5/1
  Reshape_60_3/1 -> Transpose/1
  Multiport Switch2/1 -> Compare To Constant3/1
  Bus Selector5/1 -> AdaptPointSensor2_To_Dim_60/1(ID[])  "<ID[]>"
  Bus Selector5/2 -> AdaptPointSensor2_To_Dim_60/2(Pos_ObjectPoint_CoorSys_E[x;y;z][m])  "<Pos_CoorSys_E[x;y;z][m]>"
  Bus Selector8/2 -> AdaptPointSensor3_To_Dim_60/2(Pos_ObjectPoint_CoorSys_E[x;y;z][m])  "<Pos_CoorSys_E[x;y;z][m]>"
  Multiport Switch1/1 -> Sw/3
  AdaptPointSensor3_To_Dim_60/2(Pos_ObjectPoint_CoorSys_E_Adapted[x;y;z][m]) -> Multiport Switch1/4
  AdaptPointSensor3_To_Dim_60/1(ID_Adatpted[]) -> Multiport Switch2/4
  Transpose/1 -> AnimationSignals/1

== system ASM_Traffic_new/AnimationInterface/ANIMATION_INTERFACE/Sensors/Object_Sensor_3D_Points ==
  Sw_Sensor_Selector[] : Inport
  ObjectSensor3D_1_Animation : Inport  Port=2
  ObjectSensor3D_2_Animation : Inport  Port=3
  ObjectSensor3D_3_Animation : Inport  Port=4
  Bus Selector2 : BusSelector  OutputSignals=Flag_NearestPnt_Occluded[-1|0|1],Flag_Object_In_Scope[0Out|1In],Pos_Object_NearestPnt_E[x;y;z][m]
  DownAway : Constant  Value=[zeros(MDL.Traffic.Sensors.ObjectSensor3D_Calculation.Const_Sensor_Output_Dimension.v*2,1); zeros(MDL.Traffic.Sensors.ObjectSensor3D_Calculation.Const_Sensor_Output_Dimension.v,1)-999999]
  DownAway1 : Constant  Value=[zeros(2,60-MDL.Traffic.Sensors.ObjectSensor3D_Calculation.Const_Sensor_Output_Dimension.v); zeros(1,60-MDL.Traffic.Sensors.ObjectSensor3D_Calculation.Const_Sensor_Output_Dimension.v)-999999]
  Hide_Occluded_NearestPoint[0|1] : Constant  Value=0
  Ignore_Negative : RelationalOperator  Operator===  RndMeth=Simplest  InputSameDT=off
  Mask_Hidden_Objects : Product
  Multiport Switch : MultiPortSwitch  SaturateOnIntegerOverflow=off  InputSameDT=off
  Mux : Mux  Inputs=3
  Negate : Sum  Inputs=+-
  Product : Product
  Reshape1 : Reshape  OutputDimensionality=Customize  OutputDimensions=[MDL.Traffic.Sensors.ObjectSensor3D_Calculation.Const_Sensor_Output_Dimension.v,3]
  Saturation : Saturate  UpperLimit=3  LowerLimit=1
  Saturation1 : Saturate  UpperLimit=1  LowerLimit=0
  Show_Occluded_NearestPoint[0|1]1 : Constant
  Show_Occluded_NearestPoint[0|1]2 : Constant
  Sw : MultiPortSwitch  DataPortOrder=Zero-based contiguous  Inputs=2  zeroidx=on  SaturateOnIntegerOverflow=off  InputSameDT=off
  Transpose : Math  Operator=transpose  SignedPower=on
  cc : Concatenate  Mode=Multidimensional array  ConcatenateDimension=2
  AnimationSignals : Outport  VectorParamsAs1DForOutWhenUnconnected=off
  wires:
  cc/1 -> AnimationSignals/1
  DownAway1/1 -> cc/2
  Transpose/1 -> cc/1
  Reshape1/1 -> Transpose/1
  Sw/1 -> Reshape1/1
  DownAway/1 -> Sw/2
  Bus Selector2/3 -> Sw/3  "<Pos_Object_NearestPnt_E[x;y;z][m]>"
  Multiport Switch/1 -> Bus Selector2/1
  Sw_Sensor_Selector[]/1 -> Saturation/1
  Saturation/1 -> Multiport Switch/1
  Hide_Occluded_NearestPoint[0|1]/1 -> Saturation1/1
  Saturation1/1 -> Product/1
  Mux/1 -> Sw/1
  Product/1 -> Negate/2
  Show_Occluded_NearestPoint[0|1]1/1 -> Negate/1
  Bus Selector2/1 -> Ignore_Negative/1  "<Flag_NearestPnt_Occluded[-1|0|1]>"
  Show_Occluded_NearestPoint[0|1]2/1 -> Ignore_Negative/2
  Ignore_Negative/1 -> Product/2
  Bus Selector2/2 -> Mask_Hidden_Objects/2  "<Flag_Object_In_Scope[0Out|1In]>"
  Negate/1 -> Mask_Hidden_Objects/1
  Mask_Hidden_Objects/1 -> Mux/3, Mux/1, Mux/2
  ObjectSensor3D_1_Animation/1 -> Multiport Switch/2
  ObjectSensor3D_2_Animation/1 -> Multiport Switch/3
  ObjectSensor3D_3_Animation/1 -> Multiport Switch/4

== system ASM_Traffic_new/AnimationInterface/ANIMATION_INTERFACE/Sensors/Object_Sensor_3D_RadarEffect_Points ==
  Sw_Sensor_Selector[] : Inport
  ObjectSensor3D_1_RadarEffects_Animation : Inport  Port=2
  ObjectSensor3D_2_RadarEffects_Animation : Inport  Port=3
  ObjectSensor3D_3_RadarEffects_Animation : Inport  Port=4
  AdaptPointDimensionSensor1 : Subsystem
  AdaptPointDimensionSensor2 : Subsystem
  AdaptPointDimensionSensor3 : Subsystem
  Bus Selector3 : BusSelector  OutputSignals=ID[],Pos_ObjectPoint_CoorSys_E[x;y;z][m]
  Bus Selector5 : BusSelector  OutputSignals=ID[],Pos_ObjectPoint_CoorSys_E[x;y;z][m]
  Bus Selector8 : BusSelector  OutputSignals=ID[],Pos_ObjectPoint_CoorSys_E[x;y;z][m]
  Compare To Constant3 : simulink/Logic and Bit Operations/Compare To Constant  relop=>  const=-1  OutDataTypeStr=boolean
  DownAway : Constant  Value=[zeros(60*2,1); zeros(60,1)-999999]
  Multiport Switch1 : MultiPortSwitch  SaturateOnIntegerOverflow=off  InputSameDT=off
  Multiport Switch2 : MultiPortSwitch  SaturateOnIntegerOverflow=off  InputSameDT=off
  Mux : Mux  Inputs=3
  Reshape1 : Reshape  OutputDimensionality=Customize  OutputDimensions=[60,3]
  Saturation1 : Saturate  UpperLimit=3  LowerLimit=1
  Sw : MultiPortSwitch  DataPortOrder=Zero-based contiguous  Inputs=2  zeroidx=on  SaturateOnIntegerOverflow=off  InputSameDT=off
  Transpose : Math  Operator=transpose  SignedPower=on
  AnimationSignals : Outport  VectorParamsAs1DForOutWhenUnconnected=off
  wires:
  ObjectSensor3D_1_RadarEffects_Animation/1 -> Bus Selector3/1
  ObjectSensor3D_2_RadarEffects_Animation/1 -> Bus Selector5/1
  ObjectSensor3D_3_RadarEffects_Animation/1 -> Bus Selector8/1
  Saturation1/1 -> Multiport Switch1/1, Multiport Switch2/1
  Sw_Sensor_Selector[]/1 -> Saturation1/1
  Bus Selector5/1 -> AdaptPointDimensionSensor2/1(ID[])  "<ID[]>"
  Bus Selector8/1 -> AdaptPointDimensionSensor3/1(ID[])  "<ID[]>"
  Multiport Switch2/1 -> Compare To Constant3/1
  Multiport Switch1/1 -> Sw/3
  Bus Selector3/1 -> AdaptPointDimensionSensor1/1(ID[])  "<ID[]>"
  Bus Selector3/2 -> AdaptPointDimensionSensor1/2(Pos_ObjectPoint_CoorSys_E[x;y;z][m])  "<Pos_ObjectPoint_CoorSys_E[x;y;z][m]>"
  AdaptPointDimensionSensor1/1(ID_Adatpted[]) -> Multiport Switch2/2
  AdaptPointDimensionSensor1/2(Pos_ObjectPoint_CoorSys_E_Adapted[x;y;z][m]) -> Multiport Switch1/2
  AdaptPointDimensionSensor2/1(ID_Adatpted[]) -> Multiport Switch2/3
  AdaptPointDimensionSensor2/2(Pos_ObjectPoint_CoorSys_E_Adapted[x;y;z][m]) -> Multiport Switch1/3
  Bus Selector5/2 -> AdaptPointDimensionSensor2/2(Pos_ObjectPoint_CoorSys_E[x;y;z][m])  "<Pos_ObjectPoint_CoorSys_E[x;y;z][m]>"
  AdaptPointDimensionSensor3/1(ID_Adatpted[]) -> Multiport Switch2/4
  AdaptPointDimensionSensor3/2(Pos_ObjectPoint_CoorSys_E_Adapted[x;y;z][m]) -> Multiport Switch1/4
  Compare To Constant3/1 -> Mux/3, Mux/2, Mux/1
  DownAway/1 -> Sw/2
  Sw/1 -> Reshape1/1
  Mux/1 -> Sw/1
  Reshape1/1 -> Transpose/1
  Transpose/1 -> AnimationSignals/1
  Bus Selector8/2 -> AdaptPointDimensionSensor3/2(Pos_ObjectPoint_CoorSys_E[x;y;z][m])  "<Pos_ObjectPoint_CoorSys_E[x;y;z][m]>"

== system ASM_Traffic_new/AnimationInterface/ANIMATION_INTERFACE/Sensors/Traffic_Sign_Sensor_Points ==
  ModelSignals : Inport
  Bus Selector2 : BusSelector  OutputSignals=Traffic_Sign_Valid[0|1],Pos_CoorSys_E[x;y;z][m]
  DownAway : Constant  Value=[zeros(2,MDL.Traffic.Sensors.TrafficSignSensorDyn_Calculation.Const_Sensor_Output_Dimension.v); zeros(1,MDL.Traffic.Sensors.TrafficSignSensorDyn_Calculation.Const_Sensor_Output_Dimension.v)-999999]
  DownAway1 : Constant  Value=[zeros(2,60-MDL.Traffic.Sensors.TrafficSignSensorDyn_Calculation.Const_Sensor_Output_Dimension.v); zeros(1,60-MDL.Traffic.Sensors.TrafficSignSensorDyn_Calculation.Const_Sensor_Output_Dimension.v)-999999]
  Reshape1 : Reshape  OutputDimensionality=Customize  OutputDimensions=[3,MDL.Traffic.Sensors.TrafficSignSensorDyn_Calculation.Const_Sensor_Output_Dimension.v]
  Sw : MultiPortSwitch  DataPortOrder=Zero-based contiguous  Inputs=2  zeroidx=on  SaturateOnIntegerOverflow=off  InputSameDT=off
  Trans : Math  Operator=transpose  SignedPower=on
  cc : Concatenate  NumInputs=3  Mode=Multidimensional array  ConcatenateDimension=2
  cc1 : Concatenate  Mode=Multidimensional array  ConcatenateDimension=2
  AnimationSignals : Outport  VectorParamsAs1DForOutWhenUnconnected=off
  wires:
  ModelSignals/1 -> Bus Selector2/1
  Bus Selector2/2 -> Reshape1/1  "<Pos_CoorSys_E[x;y;z][m]>"
  Bus Selector2/1 -> cc/3, cc/1, cc/2  "<Traffic_Sign_Valid[0|1]>"
  Reshape1/1 -> Sw/3
  cc/1 -> Trans/1
  Trans/1 -> Sw/1
  DownAway/1 -> Sw/2
  DownAway1/1 -> cc1/2
  Sw/1 -> cc1/1
  cc1/1 -> AnimationSignals/1

== system ASM_Traffic_new/AnimationInterface/Fellow_Lights/Coding/SwitchDelay ==
  Turnlight_L : Inport
  Turnlight_R : Inport  Port=2
  Add : Sum
  Compare To Constant : simulink/Logic and Bit Operations/Compare To Constant  relop=>  const=2  OutDataTypeStr=boolean
  Logical Operator1 : Logic  AllPortsSameDT=off  OutDataTypeStr=boolean
  Logical Operator2 : Logic  AllPortsSameDT=off  OutDataTypeStr=boolean
  Logical Operator4 : Logic  AllPortsSameDT=off  OutDataTypeStr=boolean
  Relational Operator3 : RelationalOperator  Operator=>  OutDataTypeStr=boolean  InputSameDT=off
  Switch : Switch  Criteria=u2 > Threshold  SaturateOnIntegerOverflow=off  InputSameDT=off
  Unit Delay{1..3,6} (4 alike) : UnitDelay  SampleTime=-1  HasFrameUpgradeWarning=on
  one : Constant  OutDataTypeStr=uint32
  zero : Constant  Value=0  OutDataTypeStr=uint32
  Turnlight_L_out : Outport  VectorParamsAs1DForOutWhenUnconnected=off
  Turnlight_R_out : Outport  Port=2  VectorParamsAs1DForOutWhenUnconnected=off
  wires:
  Turnlight_R/1 -> Logical Operator1/2, Unit Delay6/1
  Turnlight_L/1 -> Logical Operator1/1, Unit Delay3/1
  Logical Operator4/1 -> Turnlight_R_out/1
  Logical Operator2/1 -> Turnlight_L_out/1
  Compare To Constant/1 -> Logical Operator4/2, Logical Operator2/2
  Add/1 -> Switch/3
  Unit Delay1/1 -> Compare To Constant/1, Add/2
  one/1 -> Add/1
  Switch/1 -> Unit Delay1/1
  zero/1 -> Switch/1
  Relational Operator3/1 -> Switch/2
  Logical Operator1/1 -> Unit Delay2/1, Relational Operator3/1
  Unit Delay2/1 -> Relational Operator3/2
  Unit Delay3/1 -> Logical Operator2/1
  Unit Delay6/1 -> Logical Operator4/1

== system ASM_Traffic_new/AnimationInterface/Vehicle_Lights/Coding/SwitchDelay ==
  Turnlight_L : Inport
  Turnlight_R : Inport  Port=2
  Add : Sum
  Compare To Constant : simulink/Logic and Bit Operations/Compare To Constant  relop=>  const=2  OutDataTypeStr=boolean
  Logical Operator1 : Logic  AllPortsSameDT=off  OutDataTypeStr=boolean
  Logical Operator2 : Logic  AllPortsSameDT=off  OutDataTypeStr=boolean
  Logical Operator4 : Logic  AllPortsSameDT=off  OutDataTypeStr=boolean
  Relational Operator3 : RelationalOperator  Operator=>  OutDataTypeStr=boolean  InputSameDT=off
  Switch : Switch  Criteria=u2 > Threshold  SaturateOnIntegerOverflow=off  InputSameDT=off
  Unit Delay{1..3,6} (4 alike) : UnitDelay  SampleTime=-1  HasFrameUpgradeWarning=on
  one : Constant  OutDataTypeStr=uint32
  zero : Constant  Value=0  OutDataTypeStr=uint32
  Turnlight_L_out : Outport  VectorParamsAs1DForOutWhenUnconnected=off
  Turnlight_R_out : Outport  Port=2  VectorParamsAs1DForOutWhenUnconnected=off
  wires:
  Turnlight_R/1 -> Logical Operator1/2, Unit Delay6/1
  Turnlight_L/1 -> Logical Operator1/1, Unit Delay3/1
  Logical Operator4/1 -> Turnlight_R_out/1
  Logical Operator2/1 -> Turnlight_L_out/1
  Compare To Constant/1 -> Logical Operator4/2, Logical Operator2/2
  Add/1 -> Switch/3
  Unit Delay1/1 -> Compare To Constant/1, Add/2
  one/1 -> Add/1
  Switch/1 -> Unit Delay1/1
  zero/1 -> Switch/1
  Relational Operator3/1 -> Switch/2
  Logical Operator1/1 -> Unit Delay2/1, Relational Operator3/1
  Unit Delay2/1 -> Relational Operator3/2
  Unit Delay3/1 -> Logical Operator2/1
  Unit Delay6/1 -> Logical Operator4/1
